simulink library "sf_traffic_light_lib"  (R2025b)
settings: Solver=ode45  StartTime=0.0  StopTime=10.0  RelTol=1e-3  EnableMultiTasking=on
undefined symbols (not defined in the file or in its folder): DiscIntNeverNeededParam, GREENDELAY, LightModeType, MAXREDDELAY, MINGREENDELAY, REDDELAY, YELLOWDELAY
libraries: simulink x5
settings Model: Creator=The MathWorks, Inc.  LastModifiedBy=The MathWorks, Inc.
settings SolverCC: AlgebraicLoopSolver=TrustRegion
settings DataIOCC: LimitDataPoints=on  SaveFormat=Array  ReturnWorkspaceOutputs=off
settings OptimizationCC: ReuseModelBlockBuffer=off  LifeSpan=inf
settings DebuggingCC: UnderspecifiedInitializationDetection=Classic  MergeDetectMultiDrivingBlocksExec=none  SolverPrmCheckMsg=warning  UnconnectedInputMsg=warning  UnconnectedOutputMsg=warning  UnconnectedLineMsg=warning  StateNameClashWarn=warning  SFUnexpectedBacktrackingDiag=warning  SFNoUnconditionalDefaultTransitionDiag=warning  SFExecutionAtInitializationDiag=none  ArithmeticOperatorsInVariantConditions=warning
settings HardwareCC: ProdBitPerPointer=32.0  ProdBitPerSizeT=32.0  ProdBitPerPtrDiffT=32.0  ProdLargestAtomicFloat=None  ProdIntDivRoundTo=Undefined  ProdEndianess=Unspecified  ProdWordSize=32.0  ProdHWDeviceType=32-bit Generic
settings ModelReferenceCC: EnableRefExpFcnMdlSchedulingChecks=on  PropagateSignalLabelsOutOfModel=off
settings SFSimCC: SimUseLocalCustomCode=off  CustomCodeUndefinedFunction=UseInterfaceOnly
settings RTWCC: RTWUseLocalCustomCode=off  GPUComputeCapability=3.5
settings CodeAppCC: StateflowObjectComments=on
settings GRTTargetCC: TargetLangStandard=C89/C90 (ANSI)
settings ConfigComp: CovMetricSettings=dw  CovSaveCumulativeToWorkspaceVar=on  CovSaveSingleToWorkspaceVar=on  CovExternalEMLEnable=off

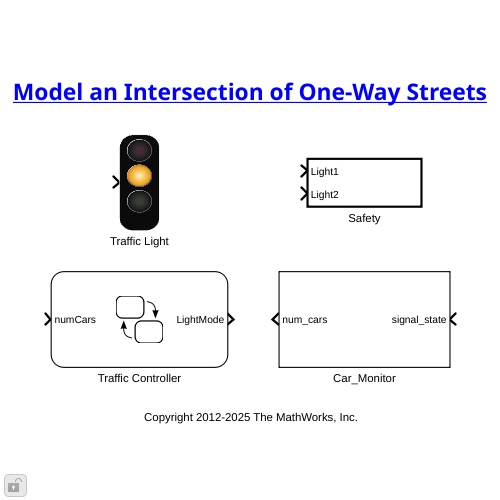
[thumbnail: Simulink's stored preview of the top-level diagram]
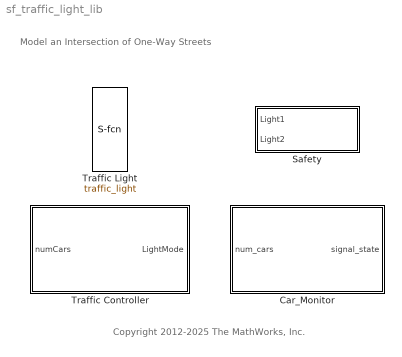
== system sf_traffic_light_lib ==
  note: Copyright 2012-2025 The MathWorks, Inc.
  note: Model an Intersection of One-Way Streets
  Car_Monitor : Subsystem
  Safety : Subsystem  TreatAsAtomicUnit=on
  Traffic Controller : Stateflow chart  TreatAsAtomicUnit=on
  Traffic Light : M-S-Function  FunctionName=traffic_light  Parameters=mode  mask{mode=LightModeType.Yellow}
      mask Display:
      | switch(mode)
      |     case LightModeType.Red
      |         image('red.jpg');
      |     case LightModeType.Green
      |         image('green.jpg');
      |     case LightModeType.Yellow
      |         image('yellow.jpg');
      |     otherwise
      |         fprintf('Error');
      | end

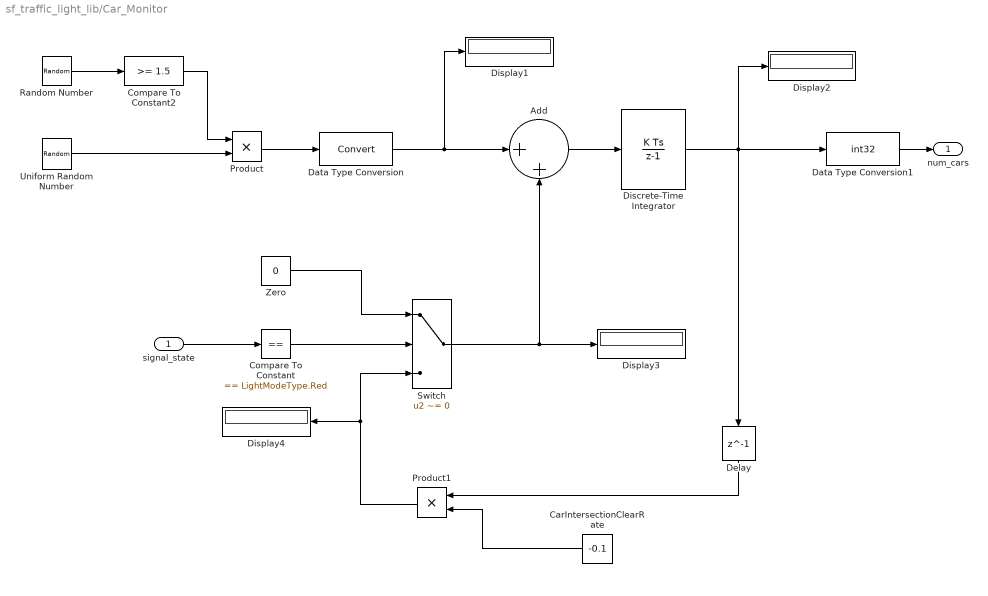
== system sf_traffic_light_lib/Car_Monitor ==
  signal_state : Inport
  Add : Sum  Inputs=|++
  CarIntersectionClearRate : Constant  Value=-0.1
  Compare To Constant : simulink/Logic and Bit Operations/Compare To Constant  relop===  const=LightModeType.Red  OutDataTypeStr=boolean  ZeroCross=off
  Compare To Constant2 : simulink/Logic and Bit Operations/Compare To Constant  relop=>=  const=1.5  OutDataTypeStr=boolean
  Data Type Conversion : DataTypeConversion  SaturateOnIntegerOverflow=off  RndMeth=Floor
  Data Type Conversion1 : DataTypeConversion  OutDataTypeStr=int32  SaturateOnIntegerOverflow=off  RndMeth=Floor
  Delay : Delay  DelayLength=1  InitialCondition=0
  Discrete-Time Integrator : DiscreteIntegrator  SampleTime=-1  LimitOutput=on  LowerSaturationLimit=0  ICPrevOutput=DiscIntNeverNeededParam  ICPrevScaledInput=DiscIntNeverNeededParam
  Display{1..4} (4 alike) : Display
  Product : Product
  Product1 : Product
  Random Number : RandomNumber  SampleTime=0.1
  Switch : Switch  Criteria=u2 ~= 0  SaturateOnIntegerOverflow=off  InputSameDT=off
  Uniform Random Number : UniformRandomNumber  Minimum=0  Maximum=5  SampleTime=0.1
  Zero : Constant  Value=0
  num_cars : Outport  VectorParamsAs1DForOutWhenUnconnected=off
  wires:
  Add/1 -> Discrete-Time Integrator/1
  Switch/1 -> Display3/1, Add/2
  Compare To Constant/1 -> Switch/2
  signal_state/1 -> Compare To Constant/1
  Discrete-Time Integrator/1 -> Data Type Conversion1/1, Delay/1, Display2/1
  Zero/1 -> Switch/1
  Product1/1 -> Display4/1, Switch/3
  Data Type Conversion1/1 -> num_cars/1
  Delay/1 -> Product1/1
  Random Number/1 -> Compare To Constant2/1
  Uniform Random Number/1 -> Product/2
  Compare To Constant2/1 -> Product/1
  Product/1 -> Data Type Conversion/1
  Data Type Conversion/1 -> Display1/1, Add/1
  CarIntersectionClearRate/1 -> Product1/2

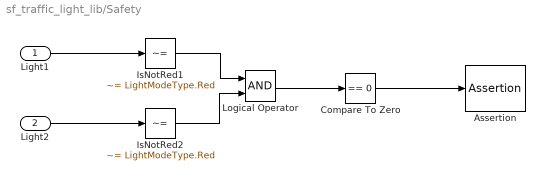
== system sf_traffic_light_lib/Safety ==
  Light1 : Inport
  Light2 : Inport  Port=2
  Assertion : Assertion
  Compare To Zero : simulink/Logic and Bit Operations/Compare To Zero  relop===  OutDataTypeStr=boolean
  IsNotRed1 : simulink/Logic and Bit Operations/Compare To Constant  relop=~=  const=LightModeType.Red  OutDataTypeStr=boolean
  IsNotRed2 : simulink/Logic and Bit Operations/Compare To Constant  relop=~=  const=LightModeType.Red  OutDataTypeStr=boolean
  Logical Operator : Logic  AllPortsSameDT=off  OutDataTypeStr=boolean
  wires:
  Light2/1 -> IsNotRed2/1
  Light1/1 -> IsNotRed1/1
  IsNotRed1/1 -> Logical Operator/1
  IsNotRed2/1 -> Logical Operator/2
  Logical Operator/1 -> Compare To Zero/1
  Compare To Zero/1 -> Assertion/1

== stateflow chart sf_traffic_light_lib/Traffic Controller ==
  state Red
    state DelayState
    state WaitForInput
    state WaitUntilSafeToChange
      du: greenLightRequested = true;
    (default) -> DelayState
    DelayState -> WaitForInput : [after(REDDELAY, sec)]
    WaitForInput -> WaitUntilSafeToChange [order 1] : [numCars > 0]
    WaitForInput -> WaitUntilSafeToChange [order 2] : [after(MAXREDDELAY,sec)]
  state Yellow
    ex:
    greenLightLocked = false;
  state Green
    en: greenLightLocked = true;
    greenLightRequested = false;
  (default) -> Red
  WaitUntilSafeToChange -> (junction 92) : [~greenLightLocked ...
      | && after(REDDELAY,sec)]
  Yellow -> Red : [after(YELLOWDELAY,sec)]
  Green -> Yellow [order 2] : [after(MINGREENDELAY, sec)...
      | && greenLightRequested]
  Green -> Yellow [order 1] : [after(GREENDELAY,sec)]
  (junction 92) -> Green
  data: numCars input; GREENDELAY parameter; MAXREDDELAY parameter; REDDELAY parameter; YELLOWDELAY parameter; MINGREENDELAY parameter; greenLightLocked data_store_memory; greenLightRequested data_store_memory; LightMode output Enum: LightModeType
